simulink model "TypeSwc"  (R2024a)
settings: Solver=FixedStepDiscrete  StartTime=0.0  StopTime=10  FixedStep=0.01  RelTol=1e-3
PreLoadFcn:
  | TypeSwc_types();
settings Model: Creator=danie  LastModifiedBy=danie
settings OptimizationCC: DefaultParameterBehavior=Inlined  EnhancedBackFolding=on  PassReuseOutputArgsAs=Individual arguments  ZeroExternalMemoryAtStartup=off  ZeroInternalMemoryAtStartup=off  OptimizeBlockOrder=speed  DifferentSizesBufferReuse=on  OptimizationCustomize=off  EfficientTunableParamExpr=on
settings DebuggingCC: ParameterTunabilityLossMsg=error
settings HardwareCC: ProdBitPerPointer=32  ProdBitPerSizeT=32  ProdBitPerPtrDiffT=32  ProdLargestAtomicInteger=Long  ProdLargestAtomicFloat=Double  ProdWordSize=32  ProdLongLongMode=on  ProdHWDeviceType=ARM Compatible->ARM Cortex-M
settings SFSimCC: SimGenImportedTypeDefs=on  MATLABDynamicMemAlloc=off
settings RTWCC: Description=AUTOSAR  SystemTargetFile=autosar.tlc  GenCodeOnly=on  GenerateMakefile=off  TemplateMakefile=ert_default_tmf  DataTypeReplacement=CDataTypesFixedWidth
settings CodeAppCC: ForceParamTrailComments=on  IgnoreCustomStorageClasses=off  MaxIdLength=63  OperatorAnnotations=on  SimulinkDataObjDesc=on  SFDataObjDesc=on  InsertBlockDesc=on
settings STFCustomTargetCC: MultiwordLength=256  ParMdlRefBuildCompliant=on  CompOptLevelCompliant=on  IncludeMdlTerminateFcn=off  CombineOutputUpdateFcns=on  SuppressErrorStatus=on  ERTCustomFileBanners=on  SupportNonFinite=off  SupportComplex=off  SupportContinuousTime=off  SupportNonInlinedSFcns=off  RemoveResetFunc=on  MATLABClassNameForMDSCustomization=Simulink.SoftwareTarget.ERTCustomization  AutosarCompliant=on  GRTInterface=off  LookupTableObjectStructAxisOrder=2,1,3,4,...  LUTObjectStructOrderEvenSpacing=Size,Table,Breakpoints  SystemTargetFile=autosar.tlc
settings ERTTargetCC: TargetLangStandard=C99 (ISO)  ConcurrentExecutionCompliant=off  IncludeMdlTerminateFcn=off  SuppressErrorStatus=on  SupportNonFinite=off  SupportComplex=off  ModelStepFunctionPrototypeControlCompliant=off  CPPClassGenCompliant=off  AutosarCompliant=on  LookupTableObjectStructAxisOrder=2,1,3,4,...  LUTObjectStructOrderEvenSpacing=Size,Table,Breakpoints  InlinedParameterPlacement=NonHierarchical  ERTCustomFileTemplate=example_file_process.tlc  BooleanTrueId=TRUE  BooleanFalseId=FALSE

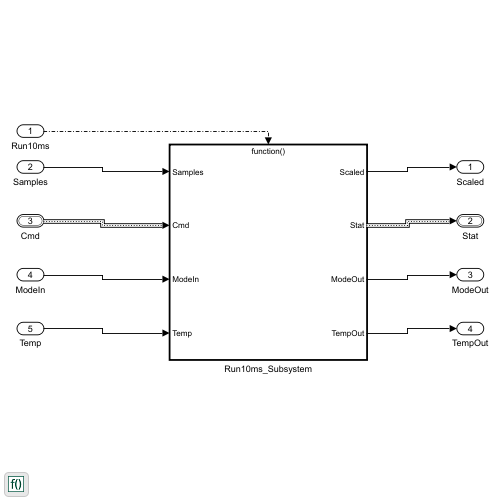
[thumbnail: Simulink's stored preview of the top-level diagram]
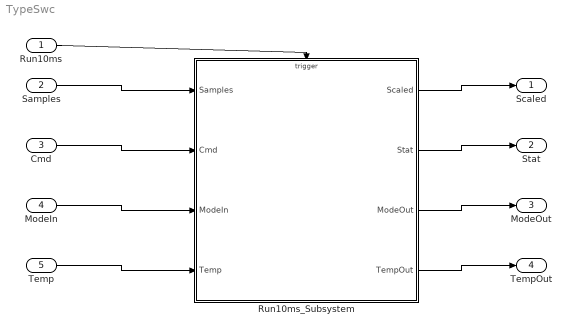
== system TypeSwc ==
  Run10ms : Inport  SampleTime=0.01  OutputFunctionCall=on
  Samples : Inport  Port=2  OutDataTypeStr=uint16  PortDimensions=4
  Cmd : Inport  Port=3  OutDataTypeStr=Bus: TypeSwc_CmdBus  PortDimensions=1  BusOutputAsStruct=on
  ModeIn : Inport  Port=4  OutDataTypeStr=Enum: TypeSwc_Mode  PortDimensions=1
  Temp : Inport  Port=5  OutDataTypeStr=fixdt(0,16,0.1,-40)  Unit=degC  PortDimensions=1
  Run10ms_Subsystem : Subsystem  TreatAsAtomicUnit=on
  Scaled : Outport  OutDataTypeStr=uint16
  Stat : Outport  Port=2  OutDataTypeStr=Bus: TypeSwc_StatBus  BusOutputAsStruct=on
  ModeOut : Outport  Port=3  OutDataTypeStr=Enum: TypeSwc_Mode
  TempOut : Outport  Port=4  OutDataTypeStr=fixdt(0,16,0.1,-40)  Unit=degC
  wires:
  Run10ms/1 -> Run10ms_Subsystem/Trigger
  Samples/1 -> Run10ms_Subsystem/1(Samples)
  Run10ms_Subsystem/1(Scaled) -> Scaled/1
  Cmd/1 -> Run10ms_Subsystem/2(Cmd)
  Run10ms_Subsystem/2(Stat) -> Stat/1
  ModeIn/1 -> Run10ms_Subsystem/3(ModeIn)
  Run10ms_Subsystem/3(ModeOut) -> ModeOut/1
  Temp/1 -> Run10ms_Subsystem/4(Temp)
  Run10ms_Subsystem/4(TempOut) -> TempOut/1

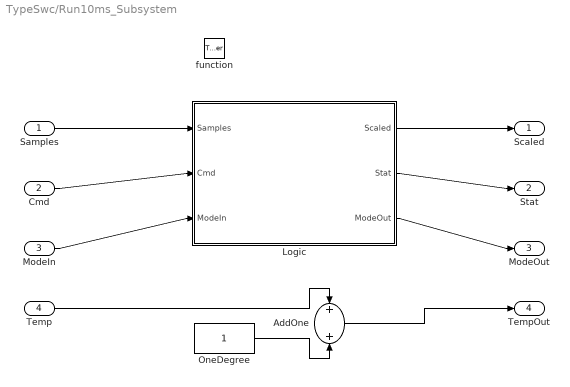
== system TypeSwc/Run10ms_Subsystem ==
  Samples : Inport
  Cmd : Inport  Port=2
  ModeIn : Inport  Port=3
  Temp : Inport  Port=4
  function : TriggerPort  TriggerType=function-call  VariantControl=(inherit)
  AddOne : Sum  OutDataTypeStr=fixdt(0,16,0.1,-40)  RndMeth=Nearest  SaturateOnIntegerOverflow=on
  Logic : MATLAB Function  TreatAsAtomicUnit=on
  OneDegree : Constant  OutDataTypeStr=fixdt(0,16,0.1,-40)
  Scaled : Outport
  Stat : Outport  Port=2
  ModeOut : Outport  Port=3
  TempOut : Outport  Port=4
  wires:
  Samples/1 -> Logic/1(Samples)
  Cmd/1 -> Logic/2(Cmd)
  ModeIn/1 -> Logic/3(ModeIn)
  Logic/1(Scaled) -> Scaled/1
  Logic/2(Stat) -> Stat/1
  Logic/3(ModeOut) -> ModeOut/1
  Temp/1 -> AddOne/1
  OneDegree/1 -> AddOne/2
  AddOne/1 -> TempOut/1

== matlab function TypeSwc/Run10ms_Subsystem/Logic ==
  data: Samples input; Scaled output uint16 size=4; Cmd input; ModeIn input; Stat output Bus: TypeSwc_StatBus; ModeOut output Enum: TypeSwc_Mode
function [Scaled, Stat, ModeOut] = Logic(Samples, Cmd, ModeIn)
%#codegen
Scaled = zeros(4, 1, 'uint16');
total = uint32(0);
largest = uint16(0);
for k = 1:4
    Scaled(k) = Samples(k) * uint16(2);   % integer arithmetic saturates
    total = total + uint32(Samples(k));
    largest = max(largest, Samples(k));
end
Stat.Sum = total;
Stat.Max = largest;
if Cmd.Enable
    Stat.Mode = Cmd.Mode;
else
    Stat.Mode = ModeIn;
end
Stat.Echo = Cmd;
if ModeIn == TypeSwc_Mode.Fault
    ModeOut = TypeSwc_Mode.Off;
else
    ModeOut = ModeIn;
end
